simulink model "Halfwave_Rectifier_Uncontrolled_RL_Load"  (R2023b)
settings: Solver=VariableStepAuto  StartTime=0.0  StopTime=1  RelTol=1e-3
libraries: spsVoltageMeasurementLib x2, spsACVoltageSourceLib x1, spsCurrentMeasurementLib x1, spsDiodeLib x1, spsSeriesRLCBranchLib x1, spspowerguiLib x1
settings Model: Creator=Anuj  LastModifiedBy=Anuj

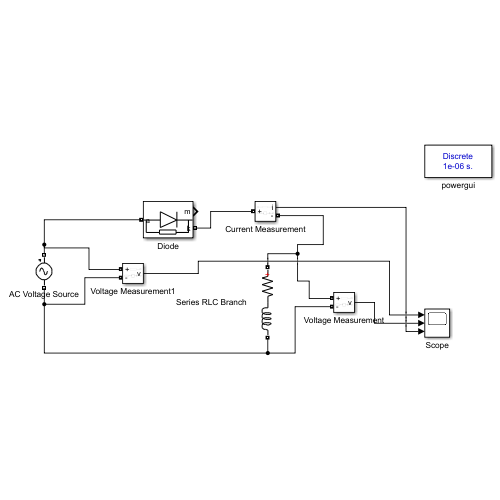
[thumbnail: Simulink's stored preview of the top-level diagram]
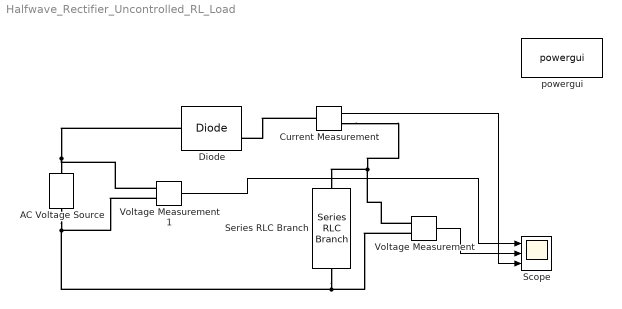
== system Halfwave_Rectifier_Uncontrolled_RL_Load ==
  "AC Voltage Source " : spsACVoltageSourceLib/AC Voltage Source  Amplitude=30*sqrt(2)  Phase=0  Frequency=50  SampleTime=0  Measurements=None  BusType=swing  Pref=10e3  Qref=0  Qmin=-inf  Qmax=+inf
  Current Measurement : spsCurrentMeasurementLib/Current Measurement  PhasorSimulation=off  OutputType=Complex  PSBequivalent=0
  Diode : spsDiodeLib/Diode  Ron=0.001  Lon=0  Vf=0.8  IC=0  UseSnubber=0  Rs=500  Cs=250e-9  Measurements=on
  Scope : Scope  NumInputPorts=3
  Series RLC Branch : spsSeriesRLCBranchLib/Series RLC Branch  LConnTagsString=__new0  RConnTagsString=__new0  BranchType=RL  Resistance=10  Inductance=10e-3  SetiL0=off  InitialCurrent=0  Capacitance=0  Setx0=off  InitialVoltage=0  Measurements=Branch voltage
  Voltage Measurement : spsVoltageMeasurementLib/Voltage Measurement  PhasorSimulation=off  OutputType=Complex  PSBequivalent=0
  Voltage Measurement1 : spsVoltageMeasurementLib/Voltage Measurement  PhasorSimulation=off  OutputType=Complex  PSBequivalent=0
  powergui : spspowerguiLib/powergui  Priority=1  SimulationMode=Discrete  SampleTime=1e-6  frequency=60  Iterations=50  frequencyindice=50  Pbase=100e6  ErrMax=1e-4  UnitsV=kV  UnitsW=MW  buscounter=0  FunctionMessages=off  echomessages=off  EnableUseOfTLC=off  CurrentSourceSwitches=off  DisableSnubberDevices=off  DisableRonSwitches=off  DisableVfSwitches=off  DisplayEquations=off  AutomaticDiscreteSolvers=off  SolverType=Tustin/Backward Euler (TBE)  Interpol=off  ExternalGateDelay=off  methode=off  Ts=100  x0status=blocks  SPID=on  SwTol=0  HookPort=off  NonlinearTolerance=1e-4  nMaxIteration=100  ContinueOnMaxIteration=off  RestoreLinks=warning  ResistiveCurrentMeasurement=off  Frange=[0:2:500]  Ylog=off  Xlog=on  ShowGrid=off  save=off  variable=ZData  structure=0  ZoomFFT=off  StartTime=0.0  cycles=1  DisplayStyle=1  fundamental=60  FreqAxis=off  MaxFrequency=1000  frequencyindicesteady=1  RmsSteady=1  display=off
  wires:
  Voltage Measurement1/1 -> Scope/1
  Voltage Measurement/1 -> Scope/2
  Current Measurement/1 -> Scope/3
  connections:
  Voltage Measurement/LConn1 -- Current Measurement/RConn1 -- Series RLC Branch/LConn1
  "AC Voltage Source "/LConn1 -- Series RLC Branch/RConn1 -- Voltage Measurement/LConn2 -- Voltage Measurement1/LConn2
  Diode/LConn1 -- Voltage Measurement1/LConn1 -- "AC Voltage Source "/RConn1
  Current Measurement/LConn1 -- Diode/RConn1
